simulink model "gtm_design_lpv"  (R2021b)
settings: Solver=VariableStepAuto  StartTime=0.0  StopTime=10  FixedStep=0.005  MaxStep=0.005  RelTol=1e-3
StopFcn:
  | MWSout=grabmws(bdroot);
  | MWSout.lastrun=datestr(now);
values from neighbouring files (symbols this model uses):
  s = tf('s')    [SingleDOF.m]    (also in main.m; mainSimple.m; newmain.m)
undefined symbols (not defined in the file or in its folder): Aero, aftfuel, aftfuel_pos, AILL, AILLC, AILR, AILRC, alpha_deg, altitude_ft, Ax_g, Ay_g, Az_g, b, beta_deg, bias, BRAKEC, Cbar, cg_pos0, cg_shift_gear, DamageCase, DamageModels, DamageOnsetTime, Earth, ELLIB, ELLIBC, ELLOB, ELLOBC, ELRIB, ELRIBC, ELROB, ELROBC, engl_ang, engl_pos, engr_ang, engr_pos, FLAPLIB, FLAPLIC, FLAPLOB, FLAPLOC, FLAPRIB, FLAPRIC, FLAPROB, FLAPROC, ft, FuelUsed_Init, fwdfuel, fwdfuel_pos, GEAR, GEARC, Inertia0, Inertia_shift_gear, Ixx_model, Iyy_model, Izz_model, KTAS, LandingGear, LengON, LinearizeModeOn, NAV_altitude_m, NAV_latitude_deg ... (+51)
libraries: simulink_extras x63, simulink_need_slupdate x30, LPVBlockLibrary x20, aerolibconvert2 x6, aerolibtransform2 x5, uavalgslib x4, UserContent_lib x3, simulink x3, robotcorelib x1, uavutilslib x1
(part 4 of 8)

== system gtm_design_lpv/GTM_T2/Aero/Basic Airframe ==
  note: The basic aerodynamics are asymmetric.
      | When the 'symmetry_on' flag is set, increments
      | from the dC3_sym aero table are added to the
      | lateral-directional coefficients (CY,Cl,Cn) to make
      | them symmetric.  When the flag is off, the gain of
      | 2.0 is applied to the increments,which effectively
      | changes the sign of the asymmetries.
  alpha : Inport
  beta : Inport  Port=2
  symmetry_on : Inport  Port=3
  AC_Params : Inport  Port=4
  Add : Sum  Inputs=+++
  AlphaLookup : PreLookup  BreakpointsData=Aero.C6_bas.alpha  IndexSearchMethod=Linear search  BeginIndexSearchUsingPreviousIndexResult=on  ExtrapMethod=Linear
  AlphaLookup1 : PreLookup  BreakpointsData=Aero.C6_bas.beta  IndexSearchMethod=Linear search  BeginIndexSearchUsingPreviousIndexResult=on  ExtrapMethod=Linear
  Assignment to Lateral : Assignment  IndexMode=Zero-based  IndexOptions=Index vector (dialog)  Indices=[1 3 5]  OutputSizes=[1 1]
  Bus Selector : BusSelector  OutputSignals=DamageCase
  Constant : Constant  Value=zeros(6,1)
  Constant1 : Constant  Value=[0:5]  OutDataTypeStr=uint32
  Constant2 : Constant  Value=[0:2]  OutDataTypeStr=uint32
  DamageEffects : Subsystem
  Data Type Conversion : DataTypeConversion  OutDataTypeStr=uint32  RndMeth=Nearest
  Gain : Gain  Gain=2
  Interpolation Using Prelookup : Interpolation_n-D  NumberOfTableDimensions=3  Table=Aero.C6_bas.data  NumSelectionDims=1
      settings: InputPortMap=u0,u1,u2,u3,u4
  Interpolation Using Prelookup1 : Interpolation_n-D  NumberOfTableDimensions=3  Table=Aero.dC3_sym.data  NumSelectionDims=1
      settings: InputPortMap=u0,u1,u2,u3,u4
  Switch : Switch  Criteria=u2 ~= 0
  C6 : Outport
  wires:
  Assignment to Lateral/1 -> Gain/1, Switch/1
  Data Type Conversion/1 -> DamageEffects/3(damage_case)
  Constant2/1 -> Interpolation Using Prelookup1/5
  Constant1/1 -> Interpolation Using Prelookup/5
  AlphaLookup1/2 -> Interpolation Using Prelookup1/4, Interpolation Using Prelookup/4
  AlphaLookup1/1 -> Interpolation Using Prelookup1/3, Interpolation Using Prelookup/3
  AlphaLookup/2 -> Interpolation Using Prelookup1/2, Interpolation Using Prelookup/2
  AlphaLookup/1 -> Interpolation Using Prelookup1/1, Interpolation Using Prelookup/1
  Bus Selector/1 -> Data Type Conversion/1  "<DamageCase>"
  AC_Params/1 -> Bus Selector/1
  DamageEffects/1(dC6_dam) -> Add/3
  beta/1 -> AlphaLookup1/1, DamageEffects/2(beta)
  alpha/1 -> AlphaLookup/1, DamageEffects/1(alpha)
  Switch/1 -> Add/2
  Add/1 -> C6/1
  symmetry_on/1 -> Switch/2
  Gain/1 -> Switch/3
  Interpolation Using Prelookup1/1 -> Assignment to Lateral/2
  Constant/1 -> Assignment to Lateral/1
  Interpolation Using Prelookup/1 -> Add/1

== system gtm_design_lpv/GTM_T2/Aero/Coefficent Evaluation ==
  C6 Body : Inport
  qbar : Inport  Port=2
  Cg : Inport  Port=3
  Cp : Inport  Port=4
  3D Vector Cross Product : Subsystem
  Demux : Demux  Outputs=[3 3]
      settings: DisplayOption=none
  Gain2 : Gain  Gain=Sref  SaturateOnIntegerOverflow=on  OutDataTypeStr=Inherit: Same as input  ParamDataTypeStr=Inherit: Same as input
  Product : Product  InputSameDT=on  SaturateOnIntegerOverflow=on  OutDataTypeStr=Inherit: Same as first input
  Reference Lengths : Gain  Gain=[b cbar b]  SaturateOnIntegerOverflow=on  OutDataTypeStr=Inherit: Same as input  ParamDataTypeStr=Inherit: Same as input
  Sum : Sum  Inputs=-+  SaturateOnIntegerOverflow=on
  Sum1 : Sum  Inputs=++|  SaturateOnIntegerOverflow=on
  Forces : Outport
  Moments : Outport  Port=2
  wires:
  3D Vector Cross Product/1(AxB) -> Sum1/1
  Sum1/1 -> Moments/1
  Reference Lengths/1 -> Sum1/2
  Demux/1 -> Forces/1, 3D Vector Cross Product/2(B)
  Demux/2 -> Reference Lengths/1
  Gain2/1 -> Demux/1
  Product/1 -> Gain2/1
  qbar/1 -> Product/2
  C6 Body/1 -> Product/1
  Cp/1 -> Sum/2
  Cg/1 -> Sum/1
  Sum/1 -> 3D Vector Cross Product/1(A)

== system gtm_design_lpv/GTM_T2/Aero/Control Surfaces ==
  note: Notes:
      | 1. Split surface effects are approximated
      | based on T2 geometry
      | Updated based on flight estimates 12/3/09
      |
      | 2. The flap model is relatively low fidelity, based
      | only on low angle of attack flight data estimates.
  alpha : Inport
  beta : Inport  Port=2  PortDimensions=1
  surfaces : Inport  Port=3
  AC_Params : Inport  Port=4
  Ailerons : Subsystem
  Bus Selector : BusSelector  OutputSignals=RUDU,RUDL
  Bus Selector13 : BusSelector  OutputSignals=GEAR
  Bus Selector14 : BusSelector  OutputSignals=DamageCase
  Bus Selector2 : BusSelector  OutputSignals=AILL,AILR
  Bus Selector3 : BusSelector  OutputSignals=SPLLIB,SPLRIB,SPLLOB,SPLROB
  Bus Selector5 : BusSelector  OutputSignals=STAB,ELLOB,ELLIB,ELRIB,ELROB
  Bus Selector9 : BusSelector  OutputSignals=FLAPLOB,FLAPLIB,FLAPRIB,FLAPROB
  Elevator/Stab1 : Subsystem
  Flaps : Subsystem
  Gear : Subsystem
  Implement Damage Models : Subsystem  mask{DamageModels=DamageModels}
      mask prompts: DamageModels "Cell Array of Damage Models"
      mask help: Implements Damage Models as gain and bias effects on selected surfaces.
      mask init:
      | SurfList={...
      |     'RUDU','RUDL',...
      |     'AILL','AILR',...
      |     'SPLLIB','SPLRIB','SPLLOB','SPLROB',...
      |     'STAB',...
      |     'ELLOB','ELLIB','ELRIB','ELROB',...
      |     'FLAPLOB','FALPLIB','FLAPRIB','FLAPROB',...
      |     'GEAR'
      |     };
      | 
      | Ncases=length(DamageModels);
      | Nsurfs=length(SurfList);
      | SurfGain=ones(Ncases,Nsurfs,6);   %Nominally unity gain, zero bias
      | 
      | %If damage case includes gain/bias on a surface adjust nominal values
      | % First damage case is "no damage".
      | for i=1:Ncases,
      |  for j=1:Nsurfs,
      |     if isfield(DamageModels{i},SurfList{j}),
      |         SurfGain(i,j,:)=DamageModels{i}.(SurfList{j}).gain*ones(1,6);
      |     end
      |  end
      | end
  Mux : Mux  Inputs=18
  Rudder : Subsystem
  Spoilers : Subsystem
  dC6 : Outport
  wires:
  Bus Selector9/4 -> Flaps/5(FLAPROB)  "<FLAPROB>"
  Bus Selector9/3 -> Flaps/4(FLAPRIB)  "<FLAPRIB>"
  Bus Selector9/2 -> Flaps/3(FLAPLIB)  "<FLAPLIB>"
  Bus Selector9/1 -> Flaps/2(FLAPLOB)  "<FLAPLOB>"
  Implement Damage Models/1(dC6) -> dC6/1
  Mux/1 -> Implement Damage Models/1(SurfVec)
  Bus Selector14/1 -> Implement Damage Models/2(damagecase)  "<DamageCase>"
  Flaps/4(RightOutb) -> Mux/17
  Flaps/3(RightInb) -> Mux/16
  Flaps/2(LeftInb) -> Mux/15
  Flaps/1(LeftOutb) -> Mux/14
  Gear/1(LandingGear) -> Mux/18
  Elevator/Stab1/5(RightOutb) -> Mux/13
  Elevator/Stab1/4(RightInb) -> Mux/12
  Elevator/Stab1/3(LeftInb) -> Mux/11
  Elevator/Stab1/2(LeftOutb) -> Mux/10
  Elevator/Stab1/1(Stab) -> Mux/9
  Spoilers/4(RightOutb) -> Mux/8
  Spoilers/3(RightInb) -> Mux/7
  Spoilers/2(LeftOutb) -> Mux/6
  Spoilers/1(LeftInb) -> Mux/5
  Ailerons/2(Right) -> Mux/4
  Ailerons/1(Left) -> Mux/3
  Rudder/2(Lower) -> Mux/2
  Rudder/1(Upper) -> Mux/1
  Bus Selector5/5 -> Elevator/Stab1/7(ELLROB)  "<ELROB>"
  Bus Selector5/4 -> Elevator/Stab1/6(ELLRIB)  "<ELRIB>"
  Bus Selector5/3 -> Elevator/Stab1/5(ELLIB)  "<ELLIB>"
  Bus Selector3/4 -> Spoilers/6(SPLROB)  "<SPLROB>"
  Bus Selector3/3 -> Spoilers/5(SPLLOB)  "<SPLLOB>"
  AC_Params/1 -> Bus Selector14/1
  alpha/1 -> [alpha]
  beta/1 -> [beta]
  surfaces/1 -> [surfaces]
  [alpha] -> Rudder/1(alpha)
  [beta] -> Rudder/2(beta)
  [surfaces] -> Bus Selector/1
  Bus Selector/1 -> Rudder/3(RUDU)  "<RUDU>"
  Bus Selector/2 -> Rudder/4(RUDL)  "<RUDL>"
  [alpha] -> Ailerons/1(alpha)
  [beta] -> Ailerons/2(beta)
  [surfaces] -> Bus Selector2/1
  Bus Selector2/1 -> Ailerons/3(AILL)  "<AILL>"
  Bus Selector2/2 -> Ailerons/4(AILR)  "<AILR>"
  [alpha] -> Spoilers/1(alpha)
  [beta] -> Spoilers/2(beta)
  [surfaces] -> Bus Selector3/1
  Bus Selector3/1 -> Spoilers/3(SPLLIB)  "<SPLLIB>"
  Bus Selector3/2 -> Spoilers/4(SPLRIB)  "<SPLRIB>"
  [beta] -> Elevator/Stab1/2(beta)
  [surfaces] -> Bus Selector5/1
  [alpha] -> Elevator/Stab1/1(alpha)
  Bus Selector5/1 -> Elevator/Stab1/3(STAB)  "<STAB>"
  Bus Selector5/2 -> Elevator/Stab1/4(ELLOB)  "<ELLOB>"
  [surfaces] -> Bus Selector9/1
  [alpha] -> Flaps/1(alpha)
  [surfaces] -> Bus Selector13/1
  [alpha] -> Gear/1(alpha)
  Bus Selector13/1 -> Gear/2(gear)  "<GEAR>"

== system gtm_design_lpv/GTM_T2/Aero/Dynamic Derviatives ==
  alpha : Inport
  beta : Inport  Port=2
  TAS : Inport  Port=3
  pqr : Inport  Port=4
  AC_Params : Inport  Port=5
  AC_Params1 : InportShadow  Port=5
  AC_Params_Dup1 : InportShadow  Port=5
  Bus Selector : BusSelector  OutputSignals=DamageCase
  Data Type Conversion : DataTypeConversion  OutDataTypeStr=uint32  RndMeth=Nearest
  Forced Oscillation with Damage Increments : Subsystem
  Merge : Merge  InitialOutput=zeros(6,1)
  Rotary Blended UnDamaged Case : Subsystem
  Switch Case : SwitchCase  CaseConditions={[1,2,3,4,5,6]}
  TAS1 : InportShadow  Port=3
  alpha_Dup1 : InportShadow
  pqr_Dup1 : InportShadow  Port=4
  dC6 : Outport
  wires:
  Forced Oscillation with Damage Increments/1(dC6) -> Merge/1
  [ndx] -> Forced Oscillation with Damage Increments/5(DamageCase)
  AC_Params1/1 -> Forced Oscillation with Damage Increments/4(AC_Params)
  pqr_Dup1/1 -> Forced Oscillation with Damage Increments/3(pqr)
  TAS1/1 -> Forced Oscillation with Damage Increments/2(TAS)
  alpha_Dup1/1 -> Forced Oscillation with Damage Increments/1(alpha)
  [ndx] -> Switch Case/1
  Data Type Conversion/1 -> [ndx]
  AC_Params_Dup1/1 -> Bus Selector/1
  Bus Selector/1 -> Data Type Conversion/1  "<DamageCase>"
  Rotary Blended UnDamaged Case/1(dC6) -> Merge/2
  Switch Case/2 -> Rotary Blended UnDamaged Case/Action
  Switch Case/1 -> Forced Oscillation with Damage Increments/Action
  Merge/1 -> dC6/1
  AC_Params/1 -> Rotary Blended UnDamaged Case/5(AC_Params)
  pqr/1 -> Rotary Blended UnDamaged Case/4(pqr)
  TAS/1 -> Rotary Blended UnDamaged Case/3(TAS)
  beta/1 -> Rotary Blended UnDamaged Case/2(beta)
  alpha/1 -> Rotary Blended UnDamaged Case/1(alpha)

== system gtm_design_lpv/GTM_T2/Aero/Label ==
  If : Inport
  Im : Inport  Port=2
  Bus Creator1 : BusCreator  Inputs=6
  Demux1 : Demux  Outputs=3
      settings: DisplayOption=none
  Demux3 : Demux  Outputs=3
      settings: DisplayOption=none
  O : Outport
  wires:
  Bus Creator1/1 -> O/1
  If/1 -> Demux1/1
  Demux1/1 -> Bus Creator1/1  "XB"
  Demux1/2 -> Bus Creator1/2  "YB"
  Demux1/3 -> Bus Creator1/3  "ZB"
  Demux3/1 -> Bus Creator1/4  "LB"
  Demux3/2 -> Bus Creator1/5  "MB"
  Demux3/3 -> Bus Creator1/6  "NB"
  Im/1 -> Demux3/1

== system gtm_design_lpv/GTM_T2/Aero/Stall Rolling Moment Asymmetry ==
  alpha : Inport
  beta : Inport  Port=2
  stall_cl_asym_enabled : Inport  Port=3
  AlphaWindow : Lookup  InputValues="[12.5   13.5   14.5]"  Table="[0  1  0]"  LookUpMeth=Interpolation-Use End Values
  Assignment to Cl : Assignment  IndexMode=Zero-based  IndexOptions=Index vector (dialog)  Indices=3  OutputSizes=[1 1]
  BetaWindow : Lookup  InputValues=[-2 -1 1 2]  Table=[0 1 1 0]  LookUpMeth=Interpolation-Use End Values
  Constant : Constant  Value=zeros(6,1)
  Product1 : Product  RndMeth=Zero
  Switch2 : Switch  Criteria=u2 > Threshold
  stall_cl_asym_coeff : Gain  Gain=0.01
  zero if disabled : Constant  Value=0
  dC6 : Outport
  wires:
  Switch2/1 -> Assignment to Cl/2
  zero if disabled/1 -> Switch2/3
  stall_cl_asym_enabled/1 -> Switch2/2
  Constant/1 -> Assignment to Cl/1
  Assignment to Cl/1 -> dC6/1
  beta/1 -> BetaWindow/1
  AlphaWindow/1 -> Product1/2
  BetaWindow/1 -> Product1/1
  Product1/1 -> stall_cl_asym_coeff/1
  alpha/1 -> AlphaWindow/1
  stall_cl_asym_coeff/1 -> Switch2/1

== system gtm_design_lpv/GTM_T2/AuxiliaryVariables/Atmos76 ==
  States : Inport
  Atmos List : Subsystem
  Bus Selector11 : BusSelector  OutputSignals=altitude
  Ground : Ground
  atmos76 : MATLAB Function  TreatAsAtomicUnit=on
  Atmos : Outport
  wires:
  Ground/1 -> atmos76/2(dt)
  Atmos List/1(O) -> Atmos/1
  States/1 -> Bus Selector11/1
  Bus Selector11/1 -> atmos76/1(z)  "<altitude>"
  atmos76/1(y) -> Atmos List/1(I)

== system gtm_design_lpv/GTM_T2/AuxiliaryVariables/Euler to DCM ==
  "Euler " : Inport
  Fcn : Fcn  Expr=u(4)*u(2)*u(6)+u(3)*u(1)
  Fcn1 : Fcn  Expr=u(3)*u(5)
  Fcn2 : Fcn  Expr=u(3)*u(2)*u(1)+u(6)*u(4)
  Fcn3 : Fcn  Expr=u(3)*u(2)*u(4)-u(6)*u(1)
  Fcn4 : Fcn  Expr=-u(2)
  Fcn5 : Fcn  Expr=u(5)*u(1)
  Fcn6 : Fcn  Expr=u(1)*u(2)*u(6)-u(3)*u(4)
  Fcn7 : Fcn  Expr=u(5)*u(6)
  Fcn8 : Fcn  Expr=u(5)*u(4)
  Mux : Mux  Inputs=2
  Mux1 : Mux  Inputs=9
  Reshape : Reshape  OutputDimensionality=Customize  OutputDimensions=[3,3]
  Trigonometric Function : Trigonometry
  Trigonometric Function1 : Trigonometry  Operator=cos
  DCM : Outport
  wires:
  "Euler "/1 -> Trigonometric Function1/1, Trigonometric Function/1
  Trigonometric Function/1 -> Mux/1
  Trigonometric Function1/1 -> Mux/2
  Mux/1 -> Fcn4/1, Fcn8/1, Fcn5/1, Fcn3/1, Fcn/1, Fcn7/1, Fcn6/1, Fcn1/1, Fcn2/1
  Mux1/1 -> Reshape/1
  Fcn7/1 -> Mux1/1
  Fcn6/1 -> Mux1/2
  Fcn/1 -> Mux1/3
  Fcn1/1 -> Mux1/4
  Fcn2/1 -> Mux1/5
  Fcn3/1 -> Mux1/6
  Fcn4/1 -> Mux1/7
  Fcn5/1 -> Mux1/8
  Fcn8/1 -> Mux1/9
  Reshape/1 -> DCM/1

== system gtm_design_lpv/GTM_T2/AuxiliaryVariables/Map 0_360 ==
  I : Inport
  Constant : Constant  Value=2*pi
  Constant1 : Constant  Value=0
  Gain : Gain  Gain=180/pi
  Sum : Sum  Inputs=|++
  ifnegadd2pi : Switch
  O : Outport
  wires:
  Gain/1 -> O/1
  Constant1/1 -> ifnegadd2pi/1
  Constant/1 -> ifnegadd2pi/3
  ifnegadd2pi/1 -> Sum/2
  Sum/1 -> Gain/1
  I/1 -> ifnegadd2pi/2, Sum/1

== system gtm_design_lpv/GTM_T2/AuxiliaryVariables/Vb Converter ==
  Vb : Inport
  Wind_b : Inport  Port=2
  Add : Sum  Inputs=+-
  Demux : Demux  Outputs=3
      settings: DisplayOption=none
  Dot Product : DotProduct  InputSameDT=on  OutDataTypeStr=Inherit: Inherit via internal rule
  Math Function : Math  Operator=sqrt  SignedPower=on  SaturateOnIntegerOverflow=on
  Product : Product  Inputs=/*  SaturateOnIntegerOverflow=on  OutDataTypeStr=Inherit: Same as first input
  Rad to Deg : Gain  Gain=180/pi  SaturateOnIntegerOverflow=on  OutDataTypeStr=Inherit: Same as input  ParamDataTypeStr=Inherit: Same as input
  Rad to Deg1 : Gain  Gain=180/pi  SaturateOnIntegerOverflow=on  OutDataTypeStr=Inherit: Same as input  ParamDataTypeStr=Inherit: Same as input
  Trigonometric Function : Trigonometry  Operator=atan2
  Trigonometric Function1 : Trigonometry  Operator=asin
  Alpha(deg) : Outport
  Beta(deg) : Outport  Port=2
  V : Outport  Port=3
  wires:
  Add/1 -> Dot Product/2, Dot Product/1, Demux/1
  Vb/1 -> Add/1
  Wind_b/1 -> Add/2
  Demux/2 -> Product/2
  Math Function/1 -> V/1, Product/1
  Product/1 -> Trigonometric Function1/1
  Demux/3 -> Trigonometric Function/1
  Demux/1 -> Trigonometric Function/2
  Dot Product/1 -> Math Function/1
  Trigonometric Function/1 -> Rad to Deg/1
  Rad to Deg/1 -> Alpha(deg)/1
  Trigonometric Function1/1 -> Rad to Deg1/1
  Rad to Deg1/1 -> Beta(deg)/1

== system gtm_design_lpv/GTM_T2/AuxiliaryVariables/VecNorm ==
  I : Inport
  Math Function2 : Math  Operator=sqrt  SignedPower=on  SaturateOnIntegerOverflow=on
  Product : Product  RndMeth=Zero
  Sum of Elements : Sum  Inputs=+
  O : Outport
  wires:
  Math Function2/1 -> O/1
  I/1 -> Product/1, Product/2
  Product/1 -> Sum of Elements/1
  Sum of Elements/1 -> Math Function2/1

== system gtm_design_lpv/GTM_T2/AuxiliaryVariables/WindShear and Xform ==
  Winds : Inport
  DCM : Inport  Port=2
  State : Inport  Port=3
  Add : Sum
  Add1 : Sum  Inputs=+-
  Bus Selector : BusSelector  OutputSignals=NorthWind,EastWind,VerticalWind  OutputAsBus=on
  Bus Selector1 : BusSelector  OutputSignals=turb_u_body,turb_v_body,turb_w_body  OutputAsBus=on
  Bus Selector11 : BusSelector  OutputSignals=altitude
  Bus to Vector : BusToVector
  Bus to Vector1 : BusToVector
  Constant : Constant  Value=WindShearOn
  Constant1 : Constant
  Constant2 : Constant  Value=runway_alt
  NED_Body : Product  Multiplication=Matrix(*)  RndMeth=Zero
  Scale : Product  Inputs=**
  Switch : Switch  Threshold=0.5
  WindShear : Subsystem
  BodyAxis Winds : Outport
  wires:
  WindShear/1(Out) -> Switch/1
  Switch/1 -> Scale/1
  Constant1/1 -> Switch/3
  Constant/1 -> Switch/2
  Add1/1 -> WindShear/1(In)
  Constant2/1 -> Add1/2
  Bus Selector11/1 -> Add1/1  "<altitude>"
  State/1 -> Bus Selector11/1
  Scale/1 -> Add/1  "SteadyWind"
  NED_Body/1 -> Scale/2
  Bus to Vector1/1 -> Add/2  "Turbulence"
  Add/1 -> BodyAxis Winds/1
  Bus Selector1/1 -> Bus to Vector1/1
  DCM/1 -> NED_Body/1
  Bus to Vector/1 -> NED_Body/2
  Bus Selector/1 -> Bus to Vector/1
  Winds/1 -> Bus Selector1/1, Bus Selector/1

== system gtm_design_lpv/GTM_T2/EOM/Aircraft 6DOF ==
  Forces : Inport  PortDimensions=6
  mass : Inport  Port=2  PortDimensions=1
  Inertia6 : Inport  Port=3  PortDimensions=6
  State : Inport  Port=4  PortDimensions=12
  3D Vector Cross Product : Subsystem
  3D Vector Cross Product1 : Subsystem
  Demux : Demux  Outputs=[3 3 3 3]
  Demux2 : Demux  Outputs=6
  Demux3 : Demux  Outputs=[3 3]
  Divide : Product  Inputs=*/
  Euler to DCM : Subsystem
  EulerDot : MATLAB Function  TreatAsAtomicUnit=on
  Form Inertia Matrix : MATLAB Function  TreatAsAtomicUnit=on
  Math Function : Math  Operator=transpose  SignedPower=on  SaturateOnIntegerOverflow=on
  Mux : Mux
  Negate Off Diag1 : Product  Inputs=**  Multiplication=Matrix(*)
  Negate Off Diag2 : Product  Inputs=**  Multiplication=Matrix(*)
  Negate Off Diag3 : Product  Inputs=**  Multiplication=Matrix(*)
  Negate Off Diag4 : Product  Inputs=**
  Sum : Sum  Inputs=-+|  SaturateOnIntegerOverflow=on
  Sum1 : Sum  Inputs=+-  SaturateOnIntegerOverflow=on
  Vlocal to LatLon : Subsystem
  Xdot : Outport
  wires:
  Negate Off Diag3/1 -> Negate Off Diag4/2
  Demux2/6 -> Form Inertia Matrix/6(Ixy)
  Demux2/5 -> Form Inertia Matrix/5(Iyz)
  Form Inertia Matrix/1(I) -> [Inertia]
  Form Inertia Matrix/2(InvI) -> [InvInertia]
  Inertia6/1 -> Demux2/1
  Demux2/4 -> Form Inertia Matrix/4(Ixz)
  Demux2/3 -> Form Inertia Matrix/3(Izz)
  Demux2/2 -> Form Inertia Matrix/2(Iyy)
  Demux2/1 -> Form Inertia Matrix/1(Ixx)
  EulerDot/1(deuler) -> Mux/4  "d/dt PhiThetaPsi"
  Sum/1 -> Mux/1  "d/dt Vb"
  Forces/1 -> Demux3/1
  Demux3/1 -> Divide/1
  mass/1 -> Divide/2
  Demux3/2 -> Sum1/1
  [Omega] -> 3D Vector Cross Product/1(A)
  [Vb] -> 3D Vector Cross Product/2(B)
  [Omega] -> Negate Off Diag1/2
  [Inertia] -> Negate Off Diag1/1
  Negate Off Diag1/1 -> 3D Vector Cross Product1/2(B)
  [Omega] -> 3D Vector Cross Product1/1(A)
  3D Vector Cross Product1/1(AxB) -> Sum1/2
  Sum1/1 -> Negate Off Diag2/2
  [InvInertia] -> Negate Off Diag2/1
  Negate Off Diag2/1 -> Mux/2  "d/dt pqr"
  [Euler] -> EulerDot/2(euler)
  [Omega] -> EulerDot/1(pqr)
  [Euler] -> Euler to DCM/1("Euler ")
  Euler to DCM/1(DCM) -> Math Function/1
  [Vb] -> Negate Off Diag3/2
  [LatLonAlt] -> Vlocal to LatLon/1(I)
  Vlocal to LatLon/1(O) -> Negate Off Diag4/1
  Negate Off Diag4/1 -> Mux/3  "d/dt LatLonAlt"
  3D Vector Cross Product/1(AxB) -> Sum/1
  Divide/1 -> Sum/2
  State/1 -> Demux/1
  Demux/1 -> [Vb]
  Demux/2 -> [Omega]
  Demux/3 -> [LatLonAlt]
  Demux/4 -> [Euler]
  Math Function/1 -> Negate Off Diag3/1
  Mux/1 -> Xdot/1

== system gtm_design_lpv/GTM_T2/EOM/Anti Windup ==
  I : Inport
  Demux : Demux  Outputs=12
      settings: DisplayOption=none
  Mux : Mux  Inputs=12
  Subsystem1 : Subsystem
      mask Display: disp('no windup 180')
  Subsystem3 : Subsystem
      mask Display: disp('no windup 180')
  Subsystem4 : Subsystem
      mask Display: disp('no windup 360')
  O : Outport
  wires:
  Mux/1 -> O/1
  Demux/11 -> Subsystem1/1(I)  "theta"
  Demux/10 -> Subsystem3/1(I)  "phi"
  Subsystem4/1(O) -> Mux/12  "psi"
  Subsystem1/1(O) -> Mux/11  "theta"
  Subsystem3/1(O) -> Mux/10  "phi"
  I/1 -> Demux/1
  Demux/1 -> Mux/1  "ub"
  Demux/2 -> Mux/2  "vb"
  Demux/3 -> Mux/3  "wb"
  Demux/4 -> Mux/4  "pb"
  Demux/5 -> Mux/5  "qb"
  Demux/6 -> Mux/6  "rb"
  Demux/7 -> Mux/7  "latitude"
  Demux/8 -> Mux/8  "longitude"
  Demux/9 -> Mux/9  "altitude"
  Demux/12 -> Subsystem4/1(I)  "psi"

== system gtm_design_lpv/GTM_T2/EOM/State Labels ==
  I : Inport
  Bus Creator : BusCreator  Inputs=12
  Demux : Demux  Outputs=12
      settings: DisplayOption=none
  O : Outport
  wires:
  Demux/12 -> Bus Creator/12  "psi"
  Demux/9 -> Bus Creator/9  "altitude"
  Demux/8 -> Bus Creator/8  "longitude"
  Demux/7 -> Bus Creator/7  "latitude"
  Demux/6 -> Bus Creator/6  "rb"
  Demux/5 -> Bus Creator/5  "qb"
  Demux/4 -> Bus Creator/4  "pb"
  Demux/3 -> Bus Creator/3  "wb"
  Demux/2 -> Bus Creator/2  "vb"
  Demux/1 -> Bus Creator/1  "ub"
  I/1 -> Demux/1
  Demux/10 -> Bus Creator/10  "phi"
  Demux/11 -> Bus Creator/11  "theta"
  Bus Creator/1 -> O/1

== system gtm_design_lpv/GTM_T2/EOM/Xdot Labels ==
  I : Inport
  Bus Creator : BusCreator  Inputs=12
  Demux : Demux  Outputs=12
      settings: DisplayOption=none
  O : Outport
  wires:
  Bus Creator/1 -> O/1
  Demux/11 -> Bus Creator/11  "theta_dot"
  Demux/10 -> Bus Creator/10  "phi_dot"
  I/1 -> Demux/1
  Demux/1 -> Bus Creator/1  "ub_dot"
  Demux/2 -> Bus Creator/2  "vb_dot"
  Demux/3 -> Bus Creator/3  "wb_dot"
  Demux/4 -> Bus Creator/4  "pb_dot"
  Demux/5 -> Bus Creator/5  "qb_dot"
  Demux/6 -> Bus Creator/6  "rb_dot"
  Demux/7 -> Bus Creator/7  "latitude_dot"
  Demux/8 -> Bus Creator/8  "longitude_dot"
  Demux/9 -> Bus Creator/9  "altitude_dot"
  Demux/12 -> Bus Creator/12  "psi_dot"

== system gtm_design_lpv/GTM_T2/Engines/3D Vector Cross Product ==
  A : Inport
  B : Inport  Port=2
  Demux : Demux  Outputs=3
      settings: DisplayOption=none
  Demux1 : Demux  Outputs=3
      settings: DisplayOption=none
  Gain : Gain  Gain=-1  SaturateOnIntegerOverflow=on  OutDataTypeStr=Inherit: Same as input  ParamDataTypeStr=Inherit: Same as input
  Ground : Ground
  Mux : Mux  Inputs=9
  Product : Product  Multiplication=Matrix(*)  SaturateOnIntegerOverflow=on  OutDataTypeStr=Inherit: Same as first input
  Reshape : Reshape  OutputDimensionality=Customize  OutputDimensions=[3,3]
  AxB : Outport
  wires:
  A/1 -> Demux/1, Gain/1
  Product/1 -> AxB/1
  Ground/1 -> Mux/1, Mux/5, Mux/9
  Gain/1 -> Demux1/1
  Demux/3 -> Mux/2
  Demux1/2 -> Mux/3
  Demux1/3 -> Mux/4
  Demux/1 -> Mux/6
  Demux/2 -> Mux/7
  Demux1/1 -> Mux/8
  Mux/1 -> Reshape/1
  Reshape/1 -> Product/1
  B/1 -> Product/2

== system gtm_design_lpv/GTM_T2/Engines/CG torque ==
  AC : Inport
  Lthrust : Inport  Port=2
  Rthrust : Inport  Port=3
  3D Vector Cross Product : Subsystem
  3D Vector Cross Product1 : Subsystem
  Bus Selector30 : BusSelector  OutputSignals=LfEng,CG,RtEng
  Sum1 : Sum  InputSameDT=on  SaturateOnIntegerOverflow=on  OutDataTypeStr=Inherit: Same as first input
  Sum6 : Sum  Inputs=+-  InputSameDT=on  SaturateOnIntegerOverflow=on  OutDataTypeStr=Inherit: Same as first input
  Sum7 : Sum  Inputs=-+  InputSameDT=on  SaturateOnIntegerOverflow=on  OutDataTypeStr=Inherit: Same as first input
  Torques : Outport
  wires:
  AC/1 -> Bus Selector30/1
  Bus Selector30/2 -> Sum7/1, Sum6/2  "<CG>"
  Lthrust/1 -> 3D Vector Cross Product1/2(B)
  Rthrust/1 -> 3D Vector Cross Product/2(B)
  Sum7/1 -> 3D Vector Cross Product/1(A)
  Sum6/1 -> 3D Vector Cross Product1/1(A)
  3D Vector Cross Product1/1(AxB) -> Sum1/1
  3D Vector Cross Product/1(AxB) -> Sum1/2
  Sum1/1 -> Torques/1
  Bus Selector30/3 -> Sum7/2  "<RtEng>"
  Bus Selector30/1 -> Sum6/1  "<LfEng>"

== system gtm_design_lpv/GTM_T2/Engines/Left_Engine Jetcat P70 ==
  Throttle : Inport
  pratio : Inport  Port=2
  tratio : Inport  Port=3
  BypassDynamics : Inport  Port=4
  qbar : Inport  Port=5
  S : Inport  Port=6
  Fuel Pump Voltage : Lookup  InputValues=fuelflow_table  Table=fuelpump_table  LookUpMeth=Interpolation-Use End Values
  Product2 : Product  RndMeth=Zero
  RPMref_2_EGT : Polyval  Coefs=Coeff_EGT
  RPMref_2_FuelFlow : Polyval  Coefs=Coeff_fuelflow
  RPMref_2_Thrust : Polyval  Coefs=Coeff_thrust
  Saturation : Saturate  UpperLimit=inf  LowerLimit=0
  Simple Ram Drag Model : MATLAB Function  TreatAsAtomicUnit=on
  Sum : Sum  Inputs=-+|
  Switch : Switch  Criteria=u2 ~= 0
  Terminator : Terminator
  Throttle Lag : Subsystem
  Throttle2 : InportShadow
  Throttle_2_RPMref : Polyval  Coefs=Coeff_throttle
  UnScale_Ref_RPM : Gain  Gain=123000/100
  angular momentum : Gain  Gain=(pi*shaft_dia^4/32) * shaft_len * density * (2*pi/60)
  Thrust (lbf) : Outport
  RPM : Outport  Port=2
  h (slg-ft^2/s) : Outport  Port=3
  Fuel Pump Voltage (V) : Outport  Port=4
  EGT (deg C) : Outport  Port=5
  Fuel Flow (lbs/min) : Outport  Port=6
  wires:
  Saturation/1 -> Thrust (lbf)/1
  Sum/1 -> Saturation/1
  Product2/1 -> Sum/2
  Simple Ram Drag Model/1(ram_drag) -> Sum/1
  S/1 -> Simple Ram Drag Model/2(S)
  qbar/1 -> Simple Ram Drag Model/1(qbar)
  Throttle2/1 -> Switch/1
  BypassDynamics/1 -> Switch/2
  Throttle Lag/1(y) -> Switch/3  "Throttle_Lag"
  Switch/1 -> Throttle_2_RPMref/1
  Throttle/1 -> Throttle Lag/1(throttle)
  Throttle_2_RPMref/1 -> RPMref_2_Thrust/1, UnScale_Ref_RPM/1, RPMref_2_EGT/1, RPMref_2_FuelFlow/1
  angular momentum/1 -> h (slg-ft^2/s)/1
  UnScale_Ref_RPM/1 -> angular momentum/1, RPM/1
  tratio/1 -> Terminator/1
  RPMref_2_Thrust/1 -> Product2/1
  RPMref_2_FuelFlow/1 -> Fuel Flow (lbs/min)/1, Fuel Pump Voltage/1
  pratio/1 -> Product2/2
  Fuel Pump Voltage/1 -> Fuel Pump Voltage (V)/1
  RPMref_2_EGT/1 -> EGT (deg C)/1

== system gtm_design_lpv/GTM_T2/Engines/Right_Engine Jetcat P70 ==
  Throttle : Inport
  pratio : Inport  Port=2
  tratio : Inport  Port=3
  BypassDynamics : Inport  Port=4
  qbar : Inport  Port=5
  S : Inport  Port=6
  Fuel Pump Voltage : Lookup  InputValues=fuelflow_table  Table=fuelpump_table  LookUpMeth=Interpolation-Use End Values
  Product2 : Product  RndMeth=Zero
  RPMref_2_EGT : Polyval  Coefs=Coeff_EGT
  RPMref_2_FuelFlow : Polyval  Coefs=Coeff_fuelflow
  RPMref_2_Thrust : Polyval  Coefs=Coeff_thrust
  Saturation : Saturate  UpperLimit=inf  LowerLimit=0
  Simple Ram Drag Model : MATLAB Function  TreatAsAtomicUnit=on
  Sum : Sum  Inputs=-+|
  Switch : Switch  Criteria=u2 ~= 0
  Terminator : Terminator
  Throttle Lag : Subsystem
  Throttle2 : InportShadow
  Throttle_2_RPMref : Polyval  Coefs=Coeff_throttle
  UnScale_Ref_RPM : Gain  Gain=123000/100
  angular momentum : Gain  Gain=(pi*shaft_dia^4/32) * shaft_len * density * (2*pi/60)
  Thrust (lbf) : Outport
  RPM : Outport  Port=2
  h (slg-ft^2/s) : Outport  Port=3
  Fuel Pump Voltage (V) : Outport  Port=4
  EGT (deg C) : Outport  Port=5
  Fuel Flow (lbs/min) : Outport  Port=6
  wires:
  Saturation/1 -> Thrust (lbf)/1
  Sum/1 -> Saturation/1
  Product2/1 -> Sum/2
  Simple Ram Drag Model/1(ram_drag) -> Sum/1
  S/1 -> Simple Ram Drag Model/2(S)
  qbar/1 -> Simple Ram Drag Model/1(qbar)
  Throttle2/1 -> Switch/1
  BypassDynamics/1 -> Switch/2
  Throttle Lag/1(y) -> Switch/3  "Throttle_Lag"
  Switch/1 -> Throttle_2_RPMref/1
  Throttle/1 -> Throttle Lag/1(throttle)
  Throttle_2_RPMref/1 -> RPMref_2_FuelFlow/1, RPMref_2_Thrust/1, UnScale_Ref_RPM/1, RPMref_2_EGT/1
  angular momentum/1 -> h (slg-ft^2/s)/1
  UnScale_Ref_RPM/1 -> angular momentum/1, RPM/1
  tratio/1 -> Terminator/1
  RPMref_2_Thrust/1 -> Product2/1
  RPMref_2_FuelFlow/1 -> Fuel Flow (lbs/min)/1, Fuel Pump Voltage/1
  pratio/1 -> Product2/2
  Fuel Pump Voltage/1 -> Fuel Pump Voltage (V)/1
  RPMref_2_EGT/1 -> EGT (deg C)/1

== system gtm_design_lpv/GTM_T2/Landing Gear/LandingGear ==
  cg : Inport  PortDimensions=3
  EulerAngles (Rad) : Inport  Port=2  PortDimensions=3
  Altitude (ft) : Inport  Port=3  PortDimensions=1
  pqr (Rad/sec) : Inport  Port=4  PortDimensions=3
  Vbody (ft/sec) : Inport  Port=5  PortDimensions=3
  Heading (Rad) : Inport  Port=6  PortDimensions=1
  Brake (0-1) : Inport  Port=7  PortDimensions=1
  Steer (deg) : Inport  Port=8  PortDimensions=1
  geardown (0/1) : Inport  Port=9  PortDimensions=1
  Data Type Conversion : DataTypeConversion  OutDataTypeStr=int32
  Euler to DCM1 : Subsystem
  Math Function : Math  Operator=transpose  SignedPower=on  SaturateOnIntegerOverflow=on
  Math Function1 : Math  Operator=transpose  SignedPower=on  SaturateOnIntegerOverflow=on
  Product : Product  Multiplication=Matrix(*)  RndMeth=Zero
  Reshape : Reshape
  S-Function1 : S-Function  FunctionName=gear_sfcn  SFunctionDeploymentMode=off  EnableBusSupport=off
  Subsystem : Subsystem
  Wheel Positions : Constant  Value=[NoseWheelPos(:);LeftMainPos(:); RightMainPos(:)];
  Wheel Positions1 : Constant  Value=SpringConst
  Wheel Positions2 : Constant  Value=DampingConst
  Wheel Positions3 : Constant  Value=MountStiffness
  Wheel Positions4 : Constant  Value=StrokeLength
  Wheel Positions5 : Constant  Value=MountDamping
  F_gear : Outport
  M_gear : Outport  Port=2
  Contact : Outport  Port=3
  wires:
  Wheel Positions5/1 -> S-Function1/5
  Math Function1/1 -> Product/1
  Vbody (ft/sec)/1 -> Product/2
  Euler to DCM1/1(DCM) -> Math Function1/1, Math Function/1
  Math Function/1 -> Reshape/1
  EulerAngles (Rad)/1 -> Euler to DCM1/1("Euler ")
  Altitude (ft)/1 -> Subsystem/1(Alt)
  geardown (0/1)/1 -> Data Type Conversion/1
  Wheel Positions/1 -> S-Function1/1
  Wheel Positions1/1 -> S-Function1/2
  Wheel Positions2/1 -> S-Function1/3
  Wheel Positions3/1 -> S-Function1/4
  Wheel Positions4/1 -> S-Function1/6
  cg/1 -> S-Function1/7
  Reshape/1 -> S-Function1/8
  Subsystem/1(cg_wrt_rwy) -> S-Function1/9
  pqr (Rad/sec)/1 -> S-Function1/10
  Product/1 -> S-Function1/11  "Vned"
  Heading (Rad)/1 -> S-Function1/12
  Brake (0-1)/1 -> S-Function1/13
  Steer (deg)/1 -> S-Function1/14
  Data Type Conversion/1 -> S-Function1/15
  S-Function1/1 -> F_gear/1
  S-Function1/2 -> M_gear/1
  S-Function1/3 -> Contact/1

== system gtm_design_lpv/GTM_T2/Sensors/Air Data ==
  EOM_State : Inport
  AuxVars : Inport  Port=2
  -50/+350 : Saturate  UpperLimit=350  LowerLimit=-50
  Bus Selector1 : BusSelector  OutputSignals=alpha,beta,qbar,tas,tratio
  Bus Selector2 : BusSelector  OutputSignals=altitude
  First Order Filter : Subsystem  mask(first order filter){tau=6}
      mask help:
      | __1__
      |  tau s+1
      |
      | First order filter  transfer function
      | with integrator IC = input  at time=0
      | If tau < Simulation Timestep, input is passed through unchanged
      | Simulation timestep must be a variable in the model/base workspace named
      | "Timestep"
      mask Help:
      | This block models a first order filter with the initial condition
      | on the integrator set to the steady state value for constant input.
      | time constant is an input
      mask Display: fprintf('  1\n--------------\n %2.1g s + 1', tau)
  Gain4 : Gain  Gain=59
  Sensor Model1 : Subsystem  mask(Sensor Model){noise_on=SensorNoise.On, sigma=SensorNoise.beta.Std, seed=878224, bias=SensorNoise.beta.Bias, scf=SensorNoise.beta.Scf}
      mask prompts: noise_on "on/off"; scf "scale factor:"
      mask help:
      | Add bias, scale factor, and white noise to a signal
      |
      | - 'on/off': 1 = noise on, 0 = noise off.
      | - 'sigma' : Standard deviation of white noise.
      | - 'seed'  : Random number seed. Generated numbers
      |   change between each simulation run, but the random number
      |   sequences do not change between Matlab sessions unless a
      |   new seed is specified.
      | - 'bias'  : Constant mean value offset of white noise.
      | - 'scale factor' : Scale factor applied to original signal.
      mask Display: disp('bias/scf/noise')
  Sensor Model2 : Subsystem  mask(Sensor Model){noise_on=SensorNoise.On, sigma=SensorNoise.KTAS.Std, seed=878654, bias=SensorNoise.KTAS.Bias, scf=SensorNoise.KTAS.Scf}
      mask prompts: noise_on "on/off"; scf "scale factor:"
      mask help:
      | Add bias, scale factor, and white noise to a signal
      |
      | - 'on/off': 1 = noise on, 0 = noise off.
      | - 'sigma' : Standard deviation of white noise.
      | - 'seed'  : Random number seed. Generated numbers
      |   change between each simulation run, but the random number
      |   sequences do not change between Matlab sessions unless a
      |   new seed is specified.
      | - 'bias'  : Constant mean value offset of white noise.
      | - 'scale factor' : Scale factor applied to original signal.
      mask Display: disp('bias/scf/noise')
  Sensor Model3 : Subsystem  mask(Sensor Model){noise_on=SensorNoise.On, sigma=SensorNoise.dyn_press.Std, seed=848234, bias=SensorNoise.dyn_press.Bias, scf=SensorNoise.dyn_press.Scf}
      mask prompts: noise_on "on/off"; scf "scale factor:"
      mask help:
      | Add bias, scale factor, and white noise to a signal
      |
      | - 'on/off': 1 = noise on, 0 = noise off.
      | - 'sigma' : Standard deviation of white noise.
      | - 'seed'  : Random number seed. Generated numbers
      |   change between each simulation run, but the random number
      |   sequences do not change between Matlab sessions unless a
      |   new seed is specified.
      | - 'bias'  : Constant mean value offset of white noise.
      | - 'scale factor' : Scale factor applied to original signal.
      mask Display: disp('bias/scf/noise')
  Sensor Model4 : Subsystem  mask(Sensor Model){noise_on=SensorNoise.On, sigma=SensorNoise.tempamb.Std, seed=878634, bias=SensorNoise.tempamb.Bias, scf=SensorNoise.tempamb.Scf}
      mask prompts: noise_on "on/off"; scf "scale factor:"
      mask help:
      | Add bias, scale factor, and white noise to a signal
      |
      | - 'on/off': 1 = noise on, 0 = noise off.
      | - 'sigma' : Standard deviation of white noise.
      | - 'seed'  : Random number seed. Generated numbers
      |   change between each simulation run, but the random number
      |   sequences do not change between Matlab sessions unless a
      |   new seed is specified.
      | - 'bias'  : Constant mean value offset of white noise.
      | - 'scale factor' : Scale factor applied to original signal.
      mask Display: disp('bias/scf/noise')
  Sensor Model5 : Subsystem  mask(Sensor Model){noise_on=SensorNoise.On, sigma=SensorNoise.alpha.Std, seed=278234, bias=SensorNoise.alpha.Bias, scf=SensorNoise.alpha.Scf}
      mask prompts: noise_on "on/off"; scf "scale factor:"
      mask help:
      | Add bias, scale factor, and white noise to a signal
      |
      | - 'on/off': 1 = noise on, 0 = noise off.
      | - 'sigma' : Standard deviation of white noise.
      | - 'seed'  : Random number seed. Generated numbers
      |   change between each simulation run, but the random number
      |   sequences do not change between Matlab sessions unless a
      |   new seed is specified.
      | - 'bias'  : Constant mean value offset of white noise.
      | - 'scale factor' : Scale factor applied to original signal.
      mask Display: disp('bias/scf/noise')
  Sensor Model6 : Subsystem  mask(Sensor Model){noise_on=SensorNoise.On, sigma=SensorNoise.baro_alt.Std, seed=878654, bias=SensorNoise.baro_alt.Bias, scf=SensorNoise.baro_alt.Scf}
      mask prompts: noise_on "on/off"; scf "scale factor:"
      mask help:
      | Add bias, scale factor, and white noise to a signal
      |
      | - 'on/off': 1 = noise on, 0 = noise off.
      | - 'sigma' : Standard deviation of white noise.
      | - 'seed'  : Random number seed. Generated numbers
      |   change between each simulation run, but the random number
      |   sequences do not change between Matlab sessions unless a
      |   new seed is specified.
      | - 'bias'  : Constant mean value offset of white noise.
      | - 'scale factor' : Scale factor applied to original signal.
      mask Display: disp('bias/scf/noise')
  pitot bus : BusCreator  Inputs=6
  AirData : Outport
  wires:
  Bus Selector1/5 -> First Order Filter/1(In)  "<tratio>"
  Sensor Model3/1(Out1) -> pitot bus/3  "qbar_psf"
  Bus Selector1/3 -> Sensor Model3/1(In1)  "<qbar>"
  pitot bus/1 -> AirData/1
  Gain4/1 -> Sensor Model4/1(In1)
  Sensor Model4/1(Out1) -> -50/+350/1
  -50/+350/1 -> pitot bus/5  "TEMPAMB_degF"
  First Order Filter/1(Out) -> Gain4/1
  Bus Selector1/1 -> Sensor Model5/1(In1)  "<alpha>"
  Bus Selector1/2 -> Sensor Model1/1(In1)  "<beta>"
  Sensor Model5/1(Out1) -> pitot bus/1  "alpha_deg"
  Sensor Model1/1(Out1) -> pitot bus/2  "beta_deg"
  Bus Selector1/4 -> Sensor Model2/1(In1)  "<tas>"
  Sensor Model2/1(Out1) -> pitot bus/4  "KTAS"
  AuxVars/1 -> Bus Selector1/1
  Bus Selector2/1 -> Sensor Model6/1(In1)  "<altitude>"
  Sensor Model6/1(Out1) -> pitot bus/6  "altitude_ft"
  EOM_State/1 -> Bus Selector2/1

== system gtm_design_lpv/GTM_T2/Sensors/Engine ECU 8 Hz ==
  Engines : Inport
  8 Hz : ZeroOrderHold  SampleTime=round(1/Timestep/8)*Timestep
  Bus Creator : BusCreator  Inputs=6
  Bus Selector : BusSelector  OutputSignals=RPML,PUMPVL,EGTL,RPMR,PUMPVR,EGTR
  RPM resolution : Quantizer  QuantizationInterval=500
      settings: AttributesFormatString=%<QuantizationInterval>
  RPM resolution1 : Quantizer  QuantizationInterval=500
      settings: AttributesFormatString=%<QuantizationInterval>
  RT : RateTransition
  Voltage resolution : Quantizer  QuantizationInterval=0.025
      settings: AttributesFormatString=%<QuantizationInterval>
  Voltage resolution1 : Quantizer  QuantizationInterval=0.025
      settings: AttributesFormatString=%<QuantizationInterval>
  deg C resolution : Quantizer  QuantizationInterval=4.6
      settings: AttributesFormatString=%<QuantizationInterval>
  deg C resolution1 : Quantizer  QuantizationInterval=4.6
      settings: AttributesFormatString=%<QuantizationInterval>
  ECU : Outport
  wires:
  8 Hz/1 -> RT/1
  Bus Creator/1 -> 8 Hz/1
  RT/1 -> ECU/1
  RPM resolution/1 -> Bus Creator/1  "RPML"
  Engines/1 -> Bus Selector/1
  deg C resolution/1 -> Bus Creator/3  "EGTL"
  RPM resolution1/1 -> Bus Creator/4  "RPMR"
  Bus Selector/1 -> RPM resolution/1  "<RPML>"
  Bus Selector/2 -> Voltage resolution/1  "<PUMPVL>"
  Bus Selector/3 -> deg C resolution/1  "<EGTL>"
  Bus Selector/4 -> RPM resolution1/1  "<RPMR>"
  Bus Selector/5 -> Voltage resolution1/1  "<PUMPVR>"
  Bus Selector/6 -> deg C resolution1/1  "<EGTR>"
  deg C resolution1/1 -> Bus Creator/6  "EGTR"
  Voltage resolution/1 -> Bus Creator/2  "PUMPVL"
  Voltage resolution1/1 -> Bus Creator/5  "PUMPVR"

== system gtm_design_lpv/GTM_T2/Sensors/MAG3 IMU ==
  AuxVars : Inport
  EOM_State : Inport  Port=2
  +/- 10g : Saturate  UpperLimit=10  LowerLimit=-10
  +/- 10g1 : Saturate  UpperLimit=10  LowerLimit=-10
  +/- 10g2 : Saturate  UpperLimit=10  LowerLimit=-10
  +/- 600 deg/sec : Saturate  UpperLimit=600  LowerLimit=-600
  +/- 600 deg/sec1 : Saturate  UpperLimit=600  LowerLimit=-600
  +/- 600 deg/sec2 : Saturate  UpperLimit=600  LowerLimit=-600
  Bus Selector2 : BusSelector  OutputSignals=Ax,Ay,Az
  Bus Selector3 : BusSelector  OutputSignals=pb,qb,rb
  MIDG bus : BusCreator  Inputs=6
  Radians to Degrees3 : simulink_extras/Transformations/Radians to Degrees
  Radians to Degrees4 : simulink_extras/Transformations/Radians to Degrees
  Radians to Degrees5 : simulink_extras/Transformations/Radians to Degrees
  Sensor Model1 : Subsystem  mask(Sensor Model){noise_on=SensorNoise.On, sigma=SensorNoise.MAG3.qdeg.Std, seed=871234, bias=SensorNoise.MAG3.qdeg.Bias, scf=SensorNoise.MAG3.qdeg.Scf}
      mask prompts: noise_on "on/off"; scf "scale factor:"
      mask help:
      | Add bias, scale factor, and white noise to a signal
      |
      | - 'on/off': 1 = noise on, 0 = noise off.
      | - 'sigma' : Standard deviation of white noise.
      | - 'seed'  : Random number seed. Generated numbers
      |   change between each simulation run, but the random number
      |   sequences do not change between Matlab sessions unless a
      |   new seed is specified.
      | - 'bias'  : Constant mean value offset of white noise.
      | - 'scale factor' : Scale factor applied to original signal.
      mask Display: disp('bias/scf/noise')
  Sensor Model2 : Subsystem  mask(Sensor Model){noise_on=SensorNoise.On, sigma=SensorNoise.MAG3.rdeg.Std, seed=878134, bias=SensorNoise.MAG3.rdeg.Bias, scf=SensorNoise.MAG3.rdeg.Scf}
      mask prompts: noise_on "on/off"; scf "scale factor:"
      mask help:
      | Add bias, scale factor, and white noise to a signal
      |
      | - 'on/off': 1 = noise on, 0 = noise off.
      | - 'sigma' : Standard deviation of white noise.
      | - 'seed'  : Random number seed. Generated numbers
      |   change between each simulation run, but the random number
      |   sequences do not change between Matlab sessions unless a
      |   new seed is specified.
      | - 'bias'  : Constant mean value offset of white noise.
      | - 'scale factor' : Scale factor applied to original signal.
      mask Display: disp('bias/scf/noise')
  Sensor Model3 : Subsystem  mask(Sensor Model){noise_on=SensorNoise.On, sigma=SensorNoise.MAG3.nxbody.Std, seed=878234, bias=SensorNoise.MAG3.nxbody.Bias, scf=SensorNoise.MAG3.nxbody.Scf}
      mask prompts: noise_on "on/off"; scf "scale factor:"
      mask help:
      | Add bias, scale factor, and white noise to a signal
      |
      | - 'on/off': 1 = noise on, 0 = noise off.
      | - 'sigma' : Standard deviation of white noise.
      | - 'seed'  : Random number seed. Generated numbers
      |   change between each simulation run, but the random number
      |   sequences do not change between Matlab sessions unless a
      |   new seed is specified.
      | - 'bias'  : Constant mean value offset of white noise.
      | - 'scale factor' : Scale factor applied to original signal.
      mask Display: disp('bias/scf/noise')
  Sensor Model4 : Subsystem  mask(Sensor Model){noise_on=SensorNoise.On, sigma=SensorNoise.MAG3.nybody.Std, seed=8782345, bias=SensorNoise.MAG3.nybody.Bias, scf=SensorNoise.MAG3.nybody.Scf}
      mask prompts: noise_on "on/off"; scf "scale factor:"
      mask help:
      | Add bias, scale factor, and white noise to a signal
      |
      | - 'on/off': 1 = noise on, 0 = noise off.
      | - 'sigma' : Standard deviation of white noise.
      | - 'seed'  : Random number seed. Generated numbers
      |   change between each simulation run, but the random number
      |   sequences do not change between Matlab sessions unless a
      |   new seed is specified.
      | - 'bias'  : Constant mean value offset of white noise.
      | - 'scale factor' : Scale factor applied to original signal.
      mask Display: disp('bias/scf/noise')
  Sensor Model5 : Subsystem  mask(Sensor Model){noise_on=SensorNoise.On, sigma=SensorNoise.MAG3.pdeg.Std, seed=878233, bias=SensorNoise.MAG3.pdeg.Bias, scf=SensorNoise.MAG3.pdeg.Scf}
      mask prompts: noise_on "on/off"; scf "scale factor:"
      mask help:
      | Add bias, scale factor, and white noise to a signal
      |
      | - 'on/off': 1 = noise on, 0 = noise off.
      | - 'sigma' : Standard deviation of white noise.
      | - 'seed'  : Random number seed. Generated numbers
      |   change between each simulation run, but the random number
      |   sequences do not change between Matlab sessions unless a
      |   new seed is specified.
      | - 'bias'  : Constant mean value offset of white noise.
      | - 'scale factor' : Scale factor applied to original signal.
      mask Display: disp('bias/scf/noise')
  Sensor Model6 : Subsystem  mask(Sensor Model){noise_on=SensorNoise.On, sigma=SensorNoise.MAG3.nzbody.Std, seed=878236, bias=SensorNoise.MAG3.nzbody.Bias, scf=SensorNoise.MAG3.nzbody.Scf}
      mask prompts: noise_on "on/off"; scf "scale factor:"
      mask help:
      | Add bias, scale factor, and white noise to a signal
      |
      | - 'on/off': 1 = noise on, 0 = noise off.
      | - 'sigma' : Standard deviation of white noise.
      | - 'seed'  : Random number seed. Generated numbers
      |   change between each simulation run, but the random number
      |   sequences do not change between Matlab sessions unless a
      |   new seed is specified.
      | - 'bias'  : Constant mean value offset of white noise.
      | - 'scale factor' : Scale factor applied to original signal.
      mask Display: disp('bias/scf/noise')
  MAG3 : Outport
  wires:
  +/- 10g2/1 -> MIDG bus/6  "Az_g"
  +/- 10g1/1 -> MIDG bus/5  "Ay_g"
  +/- 10g/1 -> MIDG bus/4  "Ax_g"
  +/- 600 deg/sec2/1 -> MIDG bus/3  "r_deg"
  +/- 600 deg/sec1/1 -> MIDG bus/2  "q_deg"
  +/- 600 deg/sec/1 -> MIDG bus/1  "p_deg"
  EOM_State/1 -> Bus Selector3/1
  Bus Selector3/1 -> Radians to Degrees3/1  "<pb>"
  Bus Selector3/2 -> Radians to Degrees4/1  "<qb>"
  Bus Selector3/3 -> Radians to Degrees5/1  "<rb>"
  Bus Selector2/1 -> Sensor Model3/1(In1)  "<Ax>"
  Bus Selector2/2 -> Sensor Model4/1(In1)  "<Ay>"
  Bus Selector2/3 -> Sensor Model6/1(In1)  "<Az>"
  Radians to Degrees3/1 -> Sensor Model5/1(In1)
  Radians to Degrees4/1 -> Sensor Model1/1(In1)
  Radians to Degrees5/1 -> Sensor Model2/1(In1)
  Sensor Model1/1(Out1) -> +/- 600 deg/sec1/1
  Sensor Model2/1(Out1) -> +/- 600 deg/sec2/1
  Sensor Model3/1(Out1) -> +/- 10g/1
  Sensor Model4/1(Out1) -> +/- 10g1/1
  Sensor Model6/1(Out1) -> +/- 10g2/1
  Sensor Model5/1(Out1) -> +/- 600 deg/sec/1
  AuxVars/1 -> Bus Selector2/1
  MIDG bus/1 -> MAG3/1
